simulink model "nodetest"  (Simulink 7.4)
settings: Solver=FixedStepDiscrete  StartTime=0.0  StopTime=10.0  FixedStep=0.1  RelTol=1e-3
libraries: dsPICdrivers x5, simulink x1
settings Model: Creator=Administrator  LastModifiedBy=Administrator
settings OptimizationCC: OptimizeModelRefInitCode=on  LifeSpan=1
settings HardwareCC: ProdBitPerInt=16  ProdEndianess=LittleEndian  ProdWordSize=16  ProdHWDeviceType=16-bit Generic
settings RTWCC: SystemTargetFile=dspic.tlc  TemplateMakefile=dspic_pic30_gcc.tmf  PostCodeGenCommand=dsPIC_Compile()  Description=Embedded Target for Microchip dsPIC (real-time)  ProcessScript=dspic_make_rtw_hook
settings CodeAppCC: IgnoreCustomStorageClasses=off
settings STFCustomTargetCC: ModelReferenceCompliant=off  IncludeMdlTerminateFcn=off  CombineOutputUpdateFcns=on  SuppressErrorStatus=on  ERTCustomFileBanners=on  SupportContinuousTime=off  SupportNonInlinedSFcns=off  SystemTargetFile=dspic.tlc
settings ERTTargetCC: MultiwordLength=2048  ModelReferenceCompliant=off  ParMdlRefBuildCompliant=off  CompOptLevelCompliant=off  IncludeMdlTerminateFcn=off  SuppressErrorStatus=on  ERTFirstTimeCompliant=off  ModelStepFunctionPrototypeControlCompliant=off  CPPClassGenCompliant=off  ExtModeMexFile=noextcomm  InlinedParameterPlacement=NonHierarchical  ERTSrcFileBannerTemplate=dsPIC_code_template.cgt  ERTHdrFileBannerTemplate=dsPIC_code_template.cgt  ERTDataSrcFileTemplate=dsPIC_code_template.cgt  ERTDataHdrFileTemplate=dsPIC_code_template.cgt  ERTCustomFileTemplate=dsPIC_main.tlc  ConvertIfToSwitch=off
settings CustomProperty: DataType=string  Value=C:\PROGRA~1\MATLAB\R2009b\bin\win32\gmake

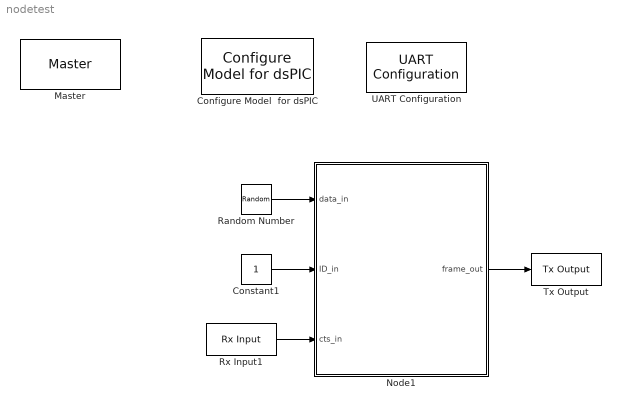
== system nodetest ==
  Configure Model  for dsPIC : dsPICdrivers/Simulink Configuration/Configure Model  for dsPIC
  Constant1 : Constant  OutDataType=fixdt(1, 16)  OutScaling=2^0  SampleTime=-1
  Master : dsPICdrivers/Master  Tag=dsPIC_MASTER  Priority=1  TimeStepType=Timer1  picType=30f4011  fcy=2.5e6  Quartz_33f=5e6  PLLActive_33f=off  fcyDesired_33f=0  tmr1="[1  2499  0]"  tmr1Info="Time Step : 0.001  ;   Error : 0%  PR1=2499"  tmr2345="[0  0  0  0]"  tmr2345cfg=[-1 -1 -1 -1]  IOautoConf=on  typePort="[ 0  0  0  0  0  0  0  0  0  0  0  0  0  0  0  0  0  0  0  0  0  0  0  0  0  0  0  0  0  0  0  0  0  0  0  0  0  0  0  0  0  0  0  0  0  5  4  0  0  0  0  0  0  0  0  0  0  0  0  0  0  0  0  0  0  0  0  0  0  0  0  0  0  0  0  0  0  0  0  0  0  0  0  0  0  0  0  0  0  0  0  0  0  0  0  0  0  0  0  0  0  0  0  0  0  0  0  0  0  0  0  0 ]"  TRIS="[ 65535  65535  65535  65535  65535  65535  65535 ]"  ADPCFG=0  MasterBusyPort=None  MasterOverloadPort=None  FOSC=HS  ClockSwitchMonitor=Both disabled  TempProtection_33f=TEMP_ON  FPBOR=BORV_20  PWRT=PWRT_OFF  MCLR=MCLR_EN  ICD=ICS_NONE  JTAGEN=JTAGEN_OFF  PowerSave=off  OverrideFcy=off  NewFcy=1e6  PR2345="[65535  65535  65535  65535]"
  Node1 : Subsystem
  Random Number : RandomNumber  Mean=4  Variance=3  SampleTime=0.1
  Rx Input1 : dsPICdrivers/Serial PORT/Rx Input  Tag=dsPIC_RX  Priority=5  UART=1  SampleTime=-1  BlockingFctChk=off  OutputDefault=0  IsPresentFlagChk=off
  Tx Output : dsPICdrivers/Serial PORT/Tx Output  Tag=dsPIC_TX  Priority=5  UART=1  OrderingInOutPopup=None
  UART Configuration : dsPICdrivers/Serial PORT/UART Configuration  Tag=dsPIC_config_UART  Priority=2  UART=1  proposed_BAUD=115200  ALT_TX_RX=on  InterruptTxWhen=When Transmit Buffer is empty  TXInterruptPri=1  TxBufferSize=32  TXEN=on  InterruptRxWhen=When Receive Buffer is full (contain 4 characters)  RXInterruptPri=2  RxBufferSize=32  BAUD=115200  UxBRG=0  Info="UxBRG = 0   ||  Real Baud : 156250   ||  % error : 35.6337  ||  max 15.625 Bytes / Step"  RealBaud=0
  wires:
  Constant1/1 -> Node1/2(ID_in)
  Random Number/1 -> Node1/1(data_in)
  Rx Input1/1 -> Node1/3(cts_in)
  Node1/1(frame_out) -> Tx Output/1

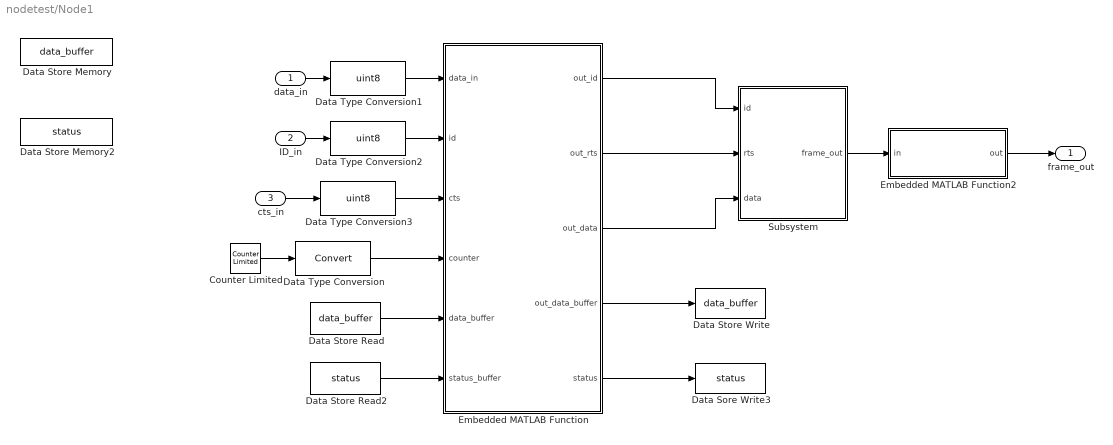
== system nodetest/Node1 ==
  data_in : Inport
  ID_in : Inport  Port=2
  cts_in : Inport  Port=3
  Counter Limited : simulink/Sources/Counter Limited  SystemSampleTime=-1  uplimit=99  tsamp=-1
  Data Sore Write3 : DataStoreWrite  DataStoreName=status  SampleTime=-1
  Data Store Memory : DataStoreMemory  DataStoreName=data_buffer  DataType=uint8  OutDataType=fixdt(1, 16)  OutScaling=2^0  OutDataTypeStr=uint8
  Data Store Memory2 : DataStoreMemory  DataStoreName=status  DataType=uint8  OutDataType=fixdt(1, 16)  OutScaling=2^0  OutDataTypeStr=uint8
  Data Store Read : DataStoreRead  DataStoreName=data_buffer  SampleTime=-1
  Data Store Read2 : DataStoreRead  DataStoreName=status  SampleTime=-1
  Data Store Write : DataStoreWrite  DataStoreName=data_buffer  SampleTime=-1
  Data Type Conversion : DataTypeConversion  OutDataType=fixdt(1, 16)  OutScaling=2^0
  Data Type Conversion1 : DataTypeConversion  OutDataTypeMode=uint8  OutDataType=fixdt(1, 16)  OutScaling=2^0  OutDataTypeStr=uint8
  Data Type Conversion2 : DataTypeConversion  OutDataTypeMode=uint8  OutDataType=fixdt(1, 16)  OutScaling=2^0  OutDataTypeStr=uint8
  Data Type Conversion3 : DataTypeConversion  OutDataTypeMode=uint8  OutDataType=fixdt(1, 16)  OutScaling=2^0  OutDataTypeStr=uint8
  Embedded MATLAB Function : Stateflow chart
  Embedded MATLAB Function2 : Stateflow chart
  Subsystem : Subsystem
  frame_out : Outport
  wires:
  Data Type Conversion3/1 -> Embedded MATLAB Function/3(cts)
  Data Type Conversion2/1 -> Embedded MATLAB Function/2(id)
  Data Type Conversion1/1 -> Embedded MATLAB Function/1(data_in)
  Embedded MATLAB Function/5(status) -> Data Sore Write3/1
  Data Store Read2/1 -> Embedded MATLAB Function/6(status_buffer)
  Data Store Read/1 -> Embedded MATLAB Function/5(data_buffer)
  Embedded MATLAB Function/4(out_data_buffer) -> Data Store Write/1
  Embedded MATLAB Function/2(out_rts) -> Subsystem/2(rts)
  Data Type Conversion/1 -> Embedded MATLAB Function/4(counter)
  Counter Limited/1 -> Data Type Conversion/1
  cts_in/1 -> Data Type Conversion3/1
  data_in/1 -> Data Type Conversion1/1
  ID_in/1 -> Data Type Conversion2/1
  Subsystem/1(frame_out) -> Embedded MATLAB Function2/1(in)
  Embedded MATLAB Function2/1(out) -> frame_out/1
  Embedded MATLAB Function/1(out_id) -> Subsystem/1(id)
  Embedded MATLAB Function/3(out_data) -> Subsystem/3(data)

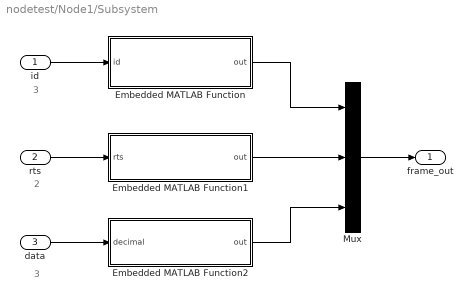
== system nodetest/Node1/Subsystem ==
  note: 3
  note: 2
  note: 3
  id : Inport  OutDataType=fixdt(1, 16)  OutScaling=2^0
  rts : Inport  Port=2  OutDataType=fixdt(1, 16)  OutScaling=2^0
  data : Inport  Port=3  OutDataType=fixdt(1, 16)  OutScaling=2^0
  Embedded MATLAB Function : Stateflow chart
  Embedded MATLAB Function1 : Stateflow chart
  Embedded MATLAB Function2 : Stateflow chart
  Mux : Mux  Inputs=3
  frame_out : Outport  OutDataType=fixdt(1, 16)  OutScaling=2^0
  wires:
  id/1 -> Embedded MATLAB Function/1(id)
  rts/1 -> Embedded MATLAB Function1/1(rts)
  data/1 -> Embedded MATLAB Function2/1(decimal)
  Embedded MATLAB Function/1(out) -> Mux/1
  Embedded MATLAB Function1/1(out) -> Mux/2
  Embedded MATLAB Function2/1(out) -> Mux/3
  Mux/1 -> frame_out/1

== matlab function Node1/Embedded MATLAB Function ==
  data: data_in input uint8; out_id output uint8; id input uint8; cts input uint8; counter input uint8; out_rts output uint8; out_data output uint8; data_buffer input uint8; out_data_buffer output uint8; status_buffer input uint8; status output uint8
function [out_id,out_rts,out_data,out_data_buffer,status] = node1_send(data_in,id,cts,counter,data_buffer,status_buffer)    %data,id,cts,counter
%#eml
rts = uint8(1);
send = false;
out_data_buffer = data_buffer; %upkeep last data_buffer value
status = status_buffer;
acknowledged = uint8(1);
data_sent = uint8(3);

if (counter == 0) 
    out_data_buffer = data_in;      %sample the input
    send = true;
    status = data_sent;
    
elseif (status ~= acknowledged)
    if (cts == id)
        status = acknowledged;
    elseif (mod(counter,10)==0)  %.1ms and no ack, resend
        send = true;
    end
end
   
if (send)
    out_id = id;
    out_rts = rts;
    out_data = out_data_buffer;
else
    out_id = uint8(0);
    out_rts = uint8(0);
    out_data = uint8(0);
end

== matlab function Node1/Subsystem/Embedded MATLAB Function ==
  data: id input double; out output double
function out = convert_id(id)
%#eml

if(id==1)
    out = [0 0 1];
elseif(id==2)
    out = [0 1 0];
elseif(id==3)
    out = [0 1 1];
elseif(id==4)
    out = [1 0 0];
else
    out = [0 0 0];
end

== matlab function Node1/Subsystem/Embedded MATLAB Function1 ==
  data: rts input double; out output double
function out = convert_rts(rts)
%#eml


if(rts==1)
    out = [0 1];
elseif(rts==2)
    out = [1 0];
elseif(rts==3)
    out = [1 1];
else
    out = [0 0];
end

== matlab function Node1/Subsystem/Embedded MATLAB Function2 ==
  data: decimal input double; out output double
function out = convert3(decimal)
%#eml

binary = zeros(1,3);
digits = uint8(3);

while(digits)
    if(mod(decimal,2))
        binary(digits) = 1;
        decimal = decimal/2 - 1;
    else
        binary(digits) = 0;
        decimal = decimal/2;
    end
    digits = digits-1;
end

out = binary;
end

== matlab function Node1/Embedded MATLAB Function2 ==
  data: in input double; out output double
function out = bin2decimal(in)
%#eml

dec = uint8(0);
for i=1:1:8
    dec = dec + in(i)*2^(8-i);
end

out = uint8(dec);
